simulink model "y2"  (R2025b)
settings: Solver=FixedStepAuto  StartTime=0.0  StopTime=10  FixedStep=0.0001  RelTol=1e-3
values from neighbouring files (symbols this model uses):
  A = [0  1; 1  1]    [adaptive_gamma_1000.mat]    (also in adaptive_gamma_10000.mat; adaptive_gamma_2000.mat; adaptive_nominal.mat; nonadaptive_nominal.mat)
undefined symbols (not defined in the file or in its folder): A_M, b, b_M, sgn
settings Model: Creator=Nickolay  LastModifiedBy=Nickolay

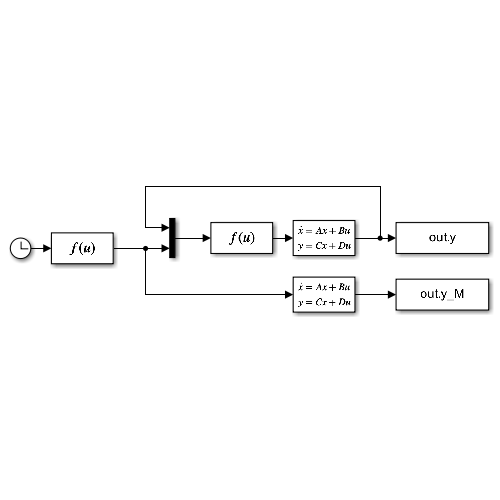
[thumbnail: Simulink's stored preview of the top-level diagram]
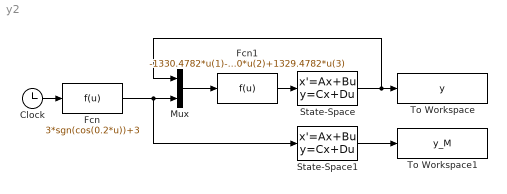
== system y2 ==
  Clock : Clock
  Fcn : Fcn  Expr=3*sgn(cos(0.2*u))+3
  Fcn1 : Fcn  Expr=-1330.4782*u(1)-73.9240*u(2)+1329.4782*u(3)
  Mux : Mux  Inputs=2
  State-Space : StateSpace  A=A  B=b  C=eye(2)  D=zeros(2,1)  InitialCondition=[0; 0]
  State-Space1 : StateSpace  A=A_M  B=b_M  C=eye(2)  D=zeros(2,1)  InitialCondition=[0; 0]
  To Workspace : ToWorkspace  VariableName=y  SaveFormat=Timeseries  SampleTime=-1
  To Workspace1 : ToWorkspace  VariableName=y_M  SaveFormat=Timeseries  SampleTime=-1
  wires:
  State-Space/1 -> Mux/1, To Workspace/1
  Fcn/1 -> Mux/2, State-Space1/1
  State-Space1/1 -> To Workspace1/1
  Clock/1 -> Fcn/1
  Fcn1/1 -> State-Space/1
  Mux/1 -> Fcn1/1
